simulink model "acf_rl_native"  (R2026b)
settings: Solver=ode4  StopTime=inf  FixedStep=3.3333333333333333e-06
InitFcn:
  | acf_select_actuator(bdroot);
model workspace (MAT data in the model file):
  acfControlVersion = 'force-observer-v1'
  acfImplementation = 'simple'
  acfLayoutVersion = 1
  p : object (value not decoded)
  pCompliant : object (value not decoded)
  pNearContact : object (value not decoded)
  pNoSprings : object (value not decoded)
  pRecommended : object (value not decoded)
symbols that are objects in the model workspace (value not decoded): p
undefined symbols (not defined in the file or in its folder): DiscIntNeverNeededParam
libraries: sl_discontinuities x1
(part 3 of 4)

== system acf_rl_native/Lateral B-S force measurement/Engineered common AA and EMA ==
  analog input : Inport
  ADC analog input filter : StateSpace  A=p.adcStudy.d.converterAnalog.A  B=p.adcStudy.d.converterAnalog.B  C=p.adcStudy.d.converterAnalog.C  D=p.adcStudy.d.converterAnalog.D  InitialCondition=((p.force.reference*(1+p.uncertainty.forceScaleX)*(-p.contact.mu*cos(p.uncertainty.forceFrameAngle_rad)-sin(p.uncertainty.forceFrameAngle_rad)+p.uncertainty.forceCrossXFromZ)))*p.adcStudy.d.converterAnalog.steadyStatePerUnitInput
  ADC clipping magnitude : Abs  SaturateOnIntegerOverflow=off
  ADC input and output noise : Sum
  ADC output noise correlation : DiscreteTransferFcn  Numerator=p.adcStudy.d.converterNoise.numerator  Denominator=p.adcStudy.d.converterNoise.denominator  SampleTime=p.adcStudy.outputSampleTime_s
  ADC range difference : Sum  Inputs=+-
  Actual ADC input range : Saturate  UpperLimit=p.adcStudy.forceAdcRange_N  LowerLimit=-(p.adcStudy.forceAdcRange_N)
  Actual ADC output samples : ZeroOrderHold  SampleTime=p.adcStudy.outputSampleTime_s
  Actual converter quantization : Quantizer  QuantizationInterval=max(p.adcStudy.forceQuantum_N,1e-15)
  Continuous analog front end : StateSpace  A=p.adcStudy.d.channels.lateral.analogA  B=p.adcStudy.d.channels.lateral.analogB  C=p.adcStudy.d.channels.lateral.analogC  D=p.adcStudy.d.channels.lateral.analogD  InitialCondition=((p.force.reference*(1+p.uncertainty.forceScaleX)*(-p.contact.mu*cos(p.uncertainty.forceFrameAngle_rad)-sin(p.uncertainty.forceFrameAngle_rad)+p.uncertainty.forceCrossXFromZ)))*p.adcStudy.d.channels.lateral.analogSteadyStatePerUnitInput
  Converter output noise RMS : Gain  Gain=p.adcStudy.forceAdcNoiseRms_N
  Fresh per-conversion EMA : DiscreteTransferFcn  Numerator=p.adcStudy.d.channels.lateral.emaNumerator  Denominator=p.adcStudy.d.channels.lateral.emaDenominator  InitialStates=(round((((p.force.reference*(1+p.uncertainty.forceScaleX)*(-p.contact.mu*cos(p.uncertainty.forceFrameAngle_rad)-sin(p.uncertainty.forceFrameAngle_rad)+p.uncertainty.forceCrossXFromZ)))+(p.adcStudy.d.lateralGravityOffset_N))/(max(p.adcStudy.forceQuantum_N,1e-15)))*(max(p.adcStudy.forceQuantum_N,1e-15))-round((p.adcStudy.d.lateralGravityOffset_N)/(max(p.adcStudy.forceQuantum_N,1e-15)))*(max(p.adcStudy.forceQuantum_N,1e-15)))*p.adcStudy.d.channels.lateral.emaSteadyStatePerUnitInput  SampleTime=p.adcStudy.outputSampleTime_s
  Independent converter output noise : RandomNumber  Seed=p.sensor.seed+2808  SampleTime=p.adcStudy.outputSampleTime_s
  Known quantized static offset : Bias  Bias=-round((p.adcStudy.d.lateralGravityOffset_N)/(max(p.adcStudy.forceQuantum_N,1e-15)))*(max(p.adcStudy.forceQuantum_N,1e-15))  SaturateOnIntegerOverflow=off
  Native converter impulse response : DiscreteTransferFcn  Numerator=p.adcStudy.d.converter.numerator  Denominator=p.adcStudy.d.converter.denominator  InitialStates=((p.force.reference*(1+p.uncertainty.forceScaleX)*(-p.contact.mu*cos(p.uncertainty.forceFrameAngle_rad)-sin(p.uncertainty.forceFrameAngle_rad)+p.uncertainty.forceCrossXFromZ)))*p.adcStudy.d.converter.steadyStatePerUnitInput  SampleTime=p.adcStudy.fineClock_s
  Restore physical static offset : Bias  Bias=p.adcStudy.d.lateralGravityOffset_N  SaturateOnIntegerOverflow=off
  conditioned output : Outport
  tag scope: lateral_adc_clip=global, lateral_adc_prequant=global
  wires:
  Actual ADC output samples/1 -> ADC input and output noise/1
  Independent converter output noise/1 -> Converter output noise RMS/1
  Converter output noise RMS/1 -> ADC output noise correlation/1
  ADC output noise correlation/1 -> ADC input and output noise/2
  ADC input and output noise/1 -> Restore physical static offset/1
  Restore physical static offset/1 -> Actual ADC input range/1, [lateral_adc_prequant], ADC range difference/1
  Actual ADC input range/1 -> Actual converter quantization/1, ADC range difference/2
  Actual converter quantization/1 -> Known quantized static offset/1
  ADC range difference/1 -> ADC clipping magnitude/1
  ADC clipping magnitude/1 -> [lateral_adc_clip]
  analog input/1 -> Continuous analog front end/1
  Continuous analog front end/1 -> ADC analog input filter/1
  ADC analog input filter/1 -> Native converter impulse response/1
  Native converter impulse response/1 -> Actual ADC output samples/1
  Known quantized static offset/1 -> Fresh per-conversion EMA/1
  Fresh per-conversion EMA/1 -> conditioned output/1

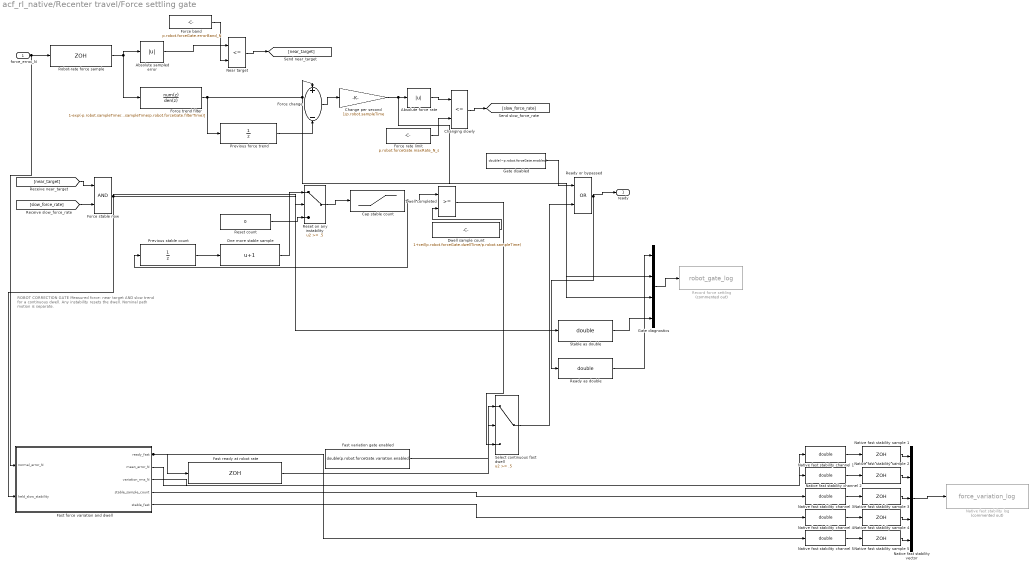
== system acf_rl_native/Recenter travel/Force settling gate ==
  note: ROBOT CORRECTION GATE
      | Measured force: near target AND slow trend for a continuous dwell.
      | Any instability resets the dwell. Nominal path motion is separate.
  force_error_N : Inport
  Absolute force rate : Abs  SaturateOnIntegerOverflow=off
  Absolute sampled error : Abs  SaturateOnIntegerOverflow=off
  Cap stable count : Saturate  UpperLimit=1+ceil(p.robot.forceGate.dwellTime/p.robot.sampleTime)  LowerLimit=0
  Change per second : Gain  Gain=1/p.robot.sampleTime
  Changing slowly : RelationalOperator  Operator=<=  OutDataTypeStr=boolean  RndMeth=Simplest  InputSameDT=off
  Dwell completed : RelationalOperator  OutDataTypeStr=boolean  RndMeth=Simplest  InputSameDT=off
  Dwell sample count : Constant  Value=1+ceil(p.robot.forceGate.dwellTime/p.robot.sampleTime)
  Fast force variation and dwell : Subsystem
  Fast ready at robot rate : ZeroOrderHold  SampleTime=p.robot.sampleTime
  Fast variation gate enabled : Constant  Value=double(p.robot.forceGate.variation.enabled)
  Force band : Constant  Value=p.robot.forceGate.errorBand_N
  Force change : Sum  Inputs=+-
  Force rate limit : Constant  Value=p.robot.forceGate.maxRate_N_s
  Force stable now : Logic  AllPortsSameDT=off  OutDataTypeStr=boolean
  Force trend filter : DiscreteTransferFcn  Numerator=1-exp(-p.robot.sampleTime/p.robot.forceGate.filterTime)  Denominator=[1 -exp(-p.robot.sampleTime/p.robot.forceGate.filterTime)]  SampleTime=p.robot.sampleTime
  Gate diagnostics : Mux
  Gate disabled : Constant  Value=double(~p.robot.forceGate.enabled)
  Native fast stability channel {1..5} (5 alike) : DataTypeConversion  OutDataTypeStr=double  SaturateOnIntegerOverflow=off  RndMeth=Floor
  Native fast stability log : ToWorkspace  Commented=on  VariableName=force_variation_log  SaveFormat=Timeseries  SampleTime=-1
  Native fast stability sample {1..5} (5 alike) : ZeroOrderHold  SampleTime=p.sim.step
  Native fast stability vector : Mux  Inputs=5
  Near target : RelationalOperator  Operator=<=  OutDataTypeStr=boolean  RndMeth=Simplest  InputSameDT=off
  One more stable sample : Bias  Bias=1  SaturateOnIntegerOverflow=off
  Previous force trend : UnitDelay  SampleTime=p.robot.sampleTime
  Previous stable count : UnitDelay  SampleTime=p.robot.sampleTime
  Ready as double : DataTypeConversion  OutDataTypeStr=double  SaturateOnIntegerOverflow=off  RndMeth=Floor
  Ready or bypassed : Logic  Operator=OR  AllPortsSameDT=off  OutDataTypeStr=boolean
  Record force settling : ToWorkspace  Commented=on  VariableName=robot_gate_log  SaveFormat=Timeseries  SampleTime=p.robot.sampleTime
  Reset count : Constant  Value=0
  Reset on any instability : Switch  Threshold=.5  SaturateOnIntegerOverflow=off  InputSameDT=off
  Robot-rate force sample : ZeroOrderHold  SampleTime=p.robot.sampleTime
  Select continuous fast dwell : Switch  Threshold=.5  SaturateOnIntegerOverflow=off  InputSameDT=off
  Stable as double : DataTypeConversion  OutDataTypeStr=double  SaturateOnIntegerOverflow=off  RndMeth=Floor
  ready : Outport
  wires:
  force_error_N/1 -> Robot-rate force sample/1, Fast force variation and dwell/1(normal_error_N)
  Robot-rate force sample/1 -> Absolute sampled error/1, Force trend filter/1
  Absolute sampled error/1 -> Near target/1
  Force band/1 -> Near target/2
  Near target/1 -> [near_target]
  Force trend filter/1 -> Force change/1, Gate diagnostics/2, Previous force trend/1
  Previous force trend/1 -> Force change/2
  Force change/1 -> Change per second/1
  Change per second/1 -> Absolute force rate/1, Gate diagnostics/3
  Absolute force rate/1 -> Changing slowly/1
  Force rate limit/1 -> Changing slowly/2
  Changing slowly/1 -> [slow_force_rate]
  [near_target] -> Force stable now/1
  [slow_force_rate] -> Force stable now/2
  Previous stable count/1 -> One more stable sample/1
  One more stable sample/1 -> Reset on any instability/1
  Force stable now/1 -> Reset on any instability/2, Stable as double/1, Fast force variation and dwell/2(held_slow_stability)
  Reset count/1 -> Reset on any instability/3
  Reset on any instability/1 -> Cap stable count/1
  Cap stable count/1 -> Previous stable count/1, Dwell completed/1
  Dwell sample count/1 -> Dwell completed/2
  Gate disabled/1 -> Ready or bypassed/1
  Ready or bypassed/1 -> ready/1, Ready as double/1
  Gate diagnostics/1 -> Record force settling/1
  Ready as double/1 -> Gate diagnostics/1
  Stable as double/1 -> Gate diagnostics/4
  Fast force variation and dwell/1(ready_fast) -> Fast ready at robot rate/1, Native fast stability channel 5/1
  Fast ready at robot rate/1 -> Select continuous fast dwell/1
  Fast variation gate enabled/1 -> Select continuous fast dwell/2
  Dwell completed/1 -> Select continuous fast dwell/3
  Select continuous fast dwell/1 -> Ready or bypassed/2
  Fast force variation and dwell/2(mean_error_N) -> Native fast stability channel 1/1
  Native fast stability channel 1/1 -> Native fast stability sample 1/1
  Native fast stability sample 1/1 -> Native fast stability vector/1
  Fast force variation and dwell/3(variation_rms_N) -> Native fast stability channel 2/1
  Native fast stability channel 2/1 -> Native fast stability sample 2/1
  Native fast stability sample 2/1 -> Native fast stability vector/2
  Fast force variation and dwell/4(stable_sample_count) -> Native fast stability channel 3/1
  Native fast stability channel 3/1 -> Native fast stability sample 3/1
  Native fast stability sample 3/1 -> Native fast stability vector/3
  Fast force variation and dwell/5(stable_fast) -> Native fast stability channel 4/1
  Native fast stability channel 4/1 -> Native fast stability sample 4/1
  Native fast stability sample 4/1 -> Native fast stability vector/4
  Native fast stability channel 5/1 -> Native fast stability sample 5/1
  Native fast stability sample 5/1 -> Native fast stability vector/5
  Native fast stability vector/1 -> Native fast stability log/1

== system acf_rl_native/S accelerometer and ADC/X engineered common AA and EMA ==
  analog input : Inport
  ADC analog input filter : StateSpace  A=p.adcStudy.d.converterAnalog.A  B=p.adcStudy.d.converterAnalog.B  C=p.adcStudy.d.converterAnalog.C  D=p.adcStudy.d.converterAnalog.D  InitialCondition=(((1+p.accel.scaleError)*(cos(p.uncertainty.accelFrameAngle_rad)*(p.mechanics.gravity*sin(p.mechanics.angle))-sin(p.uncertainty.accelFrameAngle_rad)*(p.d.g))))*p.adcStudy.d.converterAnalog.steadyStatePerUnitInput
  ADC clipping magnitude : Abs  SaturateOnIntegerOverflow=off
  ADC input and output noise : Sum
  ADC output noise correlation : DiscreteTransferFcn  Numerator=p.adcStudy.d.converterNoise.numerator  Denominator=p.adcStudy.d.converterNoise.denominator  SampleTime=p.adcStudy.outputSampleTime_s
  ADC range difference : Sum  Inputs=+-
  Actual ADC input range : Saturate  UpperLimit=min(p.adcStudy.accelerationAdcRange_g,p.accel.range_g)*p.mechanics.gravity  LowerLimit=-(min(p.adcStudy.accelerationAdcRange_g,p.accel.range_g)*p.mechanics.gravity)
  Actual ADC output samples : ZeroOrderHold  SampleTime=p.adcStudy.outputSampleTime_s
  Actual converter quantization : Quantizer  QuantizationInterval=max(p.adcStudy.accelerationQuantum_m_s2,1e-15)
  Continuous analog front end : StateSpace  A=p.adcStudy.d.channels.acceleration.analogA  B=p.adcStudy.d.channels.acceleration.analogB  C=p.adcStudy.d.channels.acceleration.analogC  D=p.adcStudy.d.channels.acceleration.analogD  InitialCondition=(((1+p.accel.scaleError)*(cos(p.uncertainty.accelFrameAngle_rad)*(p.mechanics.gravity*sin(p.mechanics.angle))-sin(p.uncertainty.accelFrameAngle_rad)*(p.d.g))))*p.adcStudy.d.channels.acceleration.analogSteadyStatePerUnitInput
  Converter output noise RMS : Gain  Gain=p.adcStudy.accelerationAdcNoiseRms_m_s2
  Fresh per-conversion EMA : DiscreteTransferFcn  Numerator=p.adcStudy.d.channels.acceleration.emaNumerator  Denominator=p.adcStudy.d.channels.acceleration.emaDenominator  InitialStates=(round(((((1+p.accel.scaleError)*(cos(p.uncertainty.accelFrameAngle_rad)*(p.mechanics.gravity*sin(p.mechanics.angle))-sin(p.uncertainty.accelFrameAngle_rad)*(p.d.g))))+(0))/(max(p.adcStudy.accelerationQuantum_m_s2,1e-15)))*(max(p.adcStudy.accelerationQuantum_m_s2,1e-15))-round((0)/(max(p.adcStudy.accelerationQuantum_m_s2,1e-15)))*(max(p.adcStudy.accelerationQuantum_m_s2,1e-15)))*p.adcStudy.d.channels.acceleration.emaSteadyStatePerUnitInput  SampleTime=p.adcStudy.outputSampleTime_s
  Independent converter output noise : RandomNumber  Seed=p.sensor.seed+3540  SampleTime=p.adcStudy.outputSampleTime_s
  Known quantized static offset : Bias  Bias=-round((0)/(max(p.adcStudy.accelerationQuantum_m_s2,1e-15)))*(max(p.adcStudy.accelerationQuantum_m_s2,1e-15))  SaturateOnIntegerOverflow=off
  Native converter impulse response : DiscreteTransferFcn  Numerator=p.adcStudy.d.converter.numerator  Denominator=p.adcStudy.d.converter.denominator  InitialStates=(((1+p.accel.scaleError)*(cos(p.uncertainty.accelFrameAngle_rad)*(p.mechanics.gravity*sin(p.mechanics.angle))-sin(p.uncertainty.accelFrameAngle_rad)*(p.d.g))))*p.adcStudy.d.converter.steadyStatePerUnitInput  SampleTime=p.adcStudy.fineClock_s
  Restore physical static offset : Bias  SaturateOnIntegerOverflow=off
  conditioned output : Outport
  tag scope: acceleration_x_adc_clip=global, acceleration_x_adc_prequant=global
  wires:
  Actual ADC output samples/1 -> ADC input and output noise/1
  Independent converter output noise/1 -> Converter output noise RMS/1
  Converter output noise RMS/1 -> ADC output noise correlation/1
  ADC output noise correlation/1 -> ADC input and output noise/2
  ADC input and output noise/1 -> Restore physical static offset/1
  Restore physical static offset/1 -> Actual ADC input range/1, [acceleration_x_adc_prequant], ADC range difference/1
  Actual ADC input range/1 -> Actual converter quantization/1, ADC range difference/2
  Actual converter quantization/1 -> Known quantized static offset/1
  ADC range difference/1 -> ADC clipping magnitude/1
  ADC clipping magnitude/1 -> [acceleration_x_adc_clip]
  analog input/1 -> Continuous analog front end/1
  Continuous analog front end/1 -> ADC analog input filter/1
  ADC analog input filter/1 -> Native converter impulse response/1
  Native converter impulse response/1 -> Actual ADC output samples/1
  Known quantized static offset/1 -> Fresh per-conversion EMA/1
  Fresh per-conversion EMA/1 -> conditioned output/1

== system acf_rl_native/S accelerometer and ADC/Z engineered common AA and EMA ==
  analog input : Inport
  ADC analog input filter : StateSpace  A=p.adcStudy.d.converterAnalog.A  B=p.adcStudy.d.converterAnalog.B  C=p.adcStudy.d.converterAnalog.C  D=p.adcStudy.d.converterAnalog.D  InitialCondition=(((1+p.accel.scaleError)*(cos(p.uncertainty.accelFrameAngle_rad)*(p.d.g)+sin(p.uncertainty.accelFrameAngle_rad)*(p.mechanics.gravity*sin(p.mechanics.angle)))))*p.adcStudy.d.converterAnalog.steadyStatePerUnitInput
  ADC clipping magnitude : Abs  SaturateOnIntegerOverflow=off
  ADC input and output noise : Sum
  ADC output noise correlation : DiscreteTransferFcn  Numerator=p.adcStudy.d.converterNoise.numerator  Denominator=p.adcStudy.d.converterNoise.denominator  SampleTime=p.adcStudy.outputSampleTime_s
  ADC range difference : Sum  Inputs=+-
  Actual ADC input range : Saturate  UpperLimit=min(p.adcStudy.accelerationAdcRange_g,p.accel.range_g)*p.mechanics.gravity  LowerLimit=-(min(p.adcStudy.accelerationAdcRange_g,p.accel.range_g)*p.mechanics.gravity)
  Actual ADC output samples : ZeroOrderHold  SampleTime=p.adcStudy.outputSampleTime_s
  Actual converter quantization : Quantizer  QuantizationInterval=max(p.adcStudy.accelerationQuantum_m_s2,1e-15)
  Continuous analog front end : StateSpace  A=p.adcStudy.d.channels.acceleration.analogA  B=p.adcStudy.d.channels.acceleration.analogB  C=p.adcStudy.d.channels.acceleration.analogC  D=p.adcStudy.d.channels.acceleration.analogD  InitialCondition=(((1+p.accel.scaleError)*(cos(p.uncertainty.accelFrameAngle_rad)*(p.d.g)+sin(p.uncertainty.accelFrameAngle_rad)*(p.mechanics.gravity*sin(p.mechanics.angle)))))*p.adcStudy.d.channels.acceleration.analogSteadyStatePerUnitInput
  Converter output noise RMS : Gain  Gain=p.adcStudy.accelerationAdcNoiseRms_m_s2
  Fresh per-conversion EMA : DiscreteTransferFcn  Numerator=p.adcStudy.d.channels.acceleration.emaNumerator  Denominator=p.adcStudy.d.channels.acceleration.emaDenominator  InitialStates=(round(((((1+p.accel.scaleError)*(cos(p.uncertainty.accelFrameAngle_rad)*(p.d.g)+sin(p.uncertainty.accelFrameAngle_rad)*(p.mechanics.gravity*sin(p.mechanics.angle)))))+(0))/(max(p.adcStudy.accelerationQuantum_m_s2,1e-15)))*(max(p.adcStudy.accelerationQuantum_m_s2,1e-15))-round((0)/(max(p.adcStudy.accelerationQuantum_m_s2,1e-15)))*(max(p.adcStudy.accelerationQuantum_m_s2,1e-15)))*p.adcStudy.d.channels.acceleration.emaSteadyStatePerUnitInput  SampleTime=p.adcStudy.outputSampleTime_s
  Independent converter output noise : RandomNumber  Seed=p.sensor.seed+3542  SampleTime=p.adcStudy.outputSampleTime_s
  Known quantized static offset : Bias  Bias=-round((0)/(max(p.adcStudy.accelerationQuantum_m_s2,1e-15)))*(max(p.adcStudy.accelerationQuantum_m_s2,1e-15))  SaturateOnIntegerOverflow=off
  Native converter impulse response : DiscreteTransferFcn  Numerator=p.adcStudy.d.converter.numerator  Denominator=p.adcStudy.d.converter.denominator  InitialStates=(((1+p.accel.scaleError)*(cos(p.uncertainty.accelFrameAngle_rad)*(p.d.g)+sin(p.uncertainty.accelFrameAngle_rad)*(p.mechanics.gravity*sin(p.mechanics.angle)))))*p.adcStudy.d.converter.steadyStatePerUnitInput  SampleTime=p.adcStudy.fineClock_s
  Restore physical static offset : Bias  SaturateOnIntegerOverflow=off
  conditioned output : Outport
  tag scope: acceleration_z_adc_clip=global, acceleration_z_adc_prequant=global
  wires:
  Actual ADC output samples/1 -> ADC input and output noise/1
  Independent converter output noise/1 -> Converter output noise RMS/1
  Converter output noise RMS/1 -> ADC output noise correlation/1
  ADC output noise correlation/1 -> ADC input and output noise/2
  ADC input and output noise/1 -> Restore physical static offset/1
  Restore physical static offset/1 -> Actual ADC input range/1, [acceleration_z_adc_prequant], ADC range difference/1
  Actual ADC input range/1 -> Actual converter quantization/1, ADC range difference/2
  Actual converter quantization/1 -> Known quantized static offset/1
  ADC range difference/1 -> ADC clipping magnitude/1
  ADC clipping magnitude/1 -> [acceleration_z_adc_clip]
  analog input/1 -> Continuous analog front end/1
  Continuous analog front end/1 -> ADC analog input filter/1
  ADC analog input filter/1 -> Native converter impulse response/1
  Native converter impulse response/1 -> Actual ADC output samples/1
  Known quantized static offset/1 -> Fresh per-conversion EMA/1
  Fresh per-conversion EMA/1 -> conditioned output/1

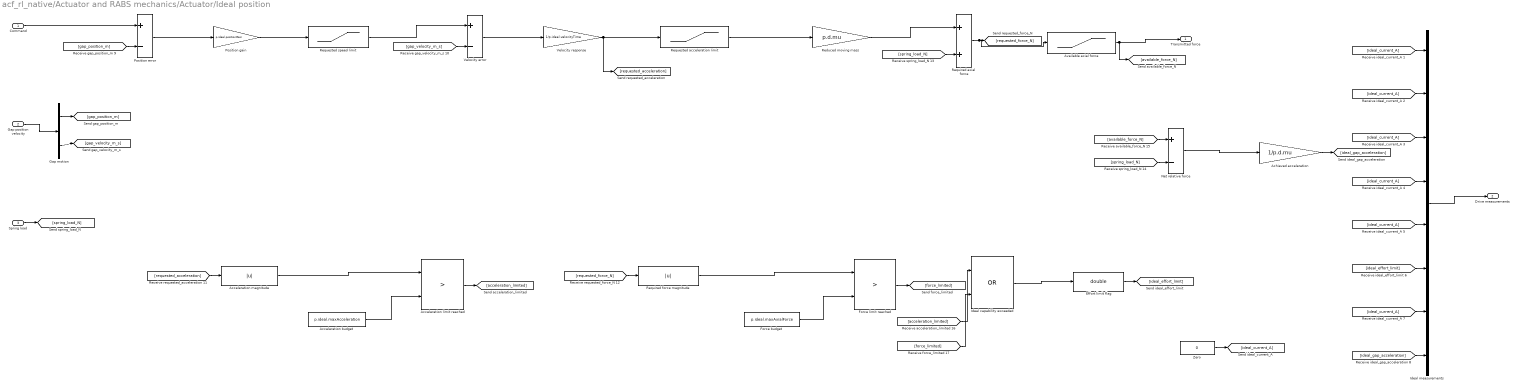
== system acf_rl_native/Actuator and RABS mechanics/Actuator/Ideal position ==
  Command : Inport
  Gap position velocity : Inport  Port=2
  Spring load : Inport  Port=3
  Acceleration budget : Constant  Value=p.ideal.maxAcceleration
  Acceleration limit reached : RelationalOperator  Operator=>  OutDataTypeStr=boolean  RndMeth=Simplest  InputSameDT=off
  Acceleration magnitude : Abs  SaturateOnIntegerOverflow=off
  Achieved acceleration : Gain  Gain=1/p.d.mu
  Available axial force : Saturate  UpperLimit=p.ideal.maxAxialForce  LowerLimit=-p.ideal.maxAxialForce
  Effort limit flag : DataTypeConversion  OutDataTypeStr=double  SaturateOnIntegerOverflow=off  RndMeth=Floor
  Force budget : Constant  Value=p.ideal.maxAxialForce
  Force limit reached : RelationalOperator  Operator=>  OutDataTypeStr=boolean  RndMeth=Simplest  InputSameDT=off
  Gap motion : Demux  Outputs=2
  Ideal capability exceeded : Logic  Operator=OR  AllPortsSameDT=off  OutDataTypeStr=boolean
  Ideal measurements : Mux  Inputs=8
  Net relative force : Sum  Inputs=+-
  Position error : Sum  Inputs=+-
  Position gain : Gain  Gain=p.ideal.positionGain
  Reduced moving mass : Gain  Gain=p.d.mu
  Requested acceleration limit : Saturate  UpperLimit=p.ideal.maxAcceleration  LowerLimit=-p.ideal.maxAcceleration
  Requested speed limit : Saturate  UpperLimit=p.ideal.maxSpeed  LowerLimit=-p.ideal.maxSpeed
  Required axial force : Sum
  Required force magnitude : Abs  SaturateOnIntegerOverflow=off
  Velocity error : Sum  Inputs=+-
  Velocity response : Gain  Gain=1/p.ideal.velocityTime
  Zero : Constant  Value=0
  Transmitted force : Outport
  Drive measurements : Outport  Port=2
  wires:
  Acceleration magnitude/1 -> Acceleration limit reached/1
  Acceleration budget/1 -> Acceleration limit reached/2
  [requested_acceleration] -> Acceleration magnitude/1
  Net relative force/1 -> Achieved acceleration/1
  Required axial force/1 -> Available axial force/1, [requested_force_N]
  Ideal capability exceeded/1 -> Effort limit flag/1
  Required force magnitude/1 -> Force limit reached/1
  Force budget/1 -> Force limit reached/2
  Gap position velocity/1 -> Gap motion/1
  [acceleration_limited] -> Ideal capability exceeded/1
  [force_limited] -> Ideal capability exceeded/2
  [ideal_current_A] -> Ideal measurements/1
  [ideal_current_A] -> Ideal measurements/2
  [ideal_current_A] -> Ideal measurements/3
  [ideal_current_A] -> Ideal measurements/4
  [ideal_current_A] -> Ideal measurements/5
  [ideal_effort_limit] -> Ideal measurements/6
  [ideal_current_A] -> Ideal measurements/7
  [ideal_gap_acceleration] -> Ideal measurements/8
  [available_force_N] -> Net relative force/1
  [spring_load_N] -> Net relative force/2
  Command/1 -> Position error/1
  [gap_position_m] -> Position error/2
  Position error/1 -> Position gain/1
  Requested acceleration limit/1 -> Reduced moving mass/1
  Velocity response/1 -> Requested acceleration limit/1, [requested_acceleration]
  Position gain/1 -> Requested speed limit/1
  Reduced moving mass/1 -> Required axial force/1
  [spring_load_N] -> Required axial force/2
  [requested_force_N] -> Required force magnitude/1
  Acceleration limit reached/1 -> [acceleration_limited]
  Available axial force/1 -> [available_force_N], Transmitted force/1
  Force limit reached/1 -> [force_limited]
  Gap motion/1 -> [gap_position_m]
  Gap motion/2 -> [gap_velocity_m_s]
  Zero/1 -> [ideal_current_A]
  Effort limit flag/1 -> [ideal_effort_limit]
  Achieved acceleration/1 -> [ideal_gap_acceleration]
  Spring load/1 -> [spring_load_N]
  Requested speed limit/1 -> Velocity error/1
  [gap_velocity_m_s] -> Velocity error/2
  Velocity error/1 -> Velocity response/1
  Ideal measurements/1 -> Drive measurements/1

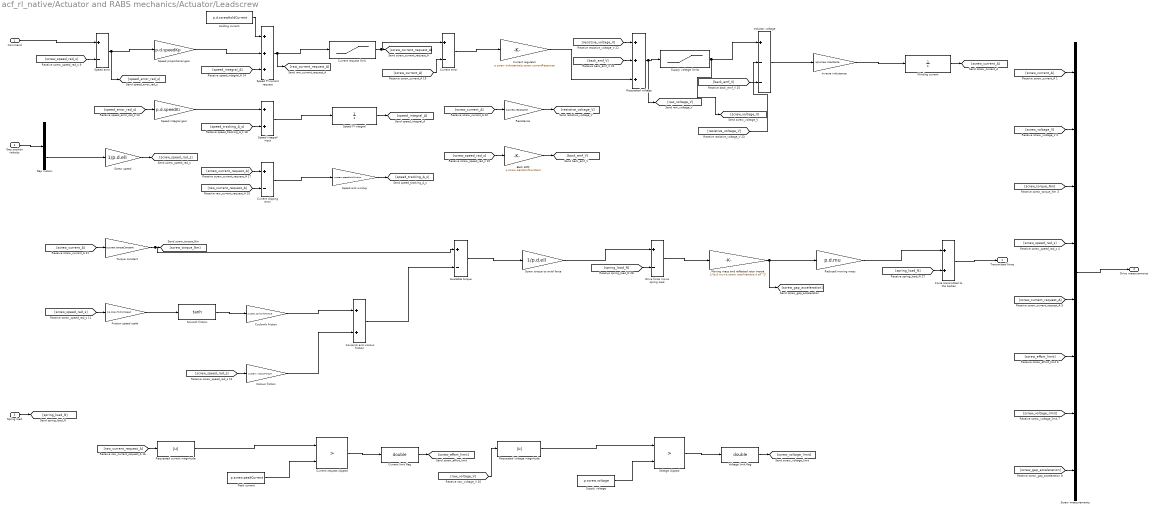
== system acf_rl_native/Actuator and RABS mechanics/Actuator/Leadscrew ==
  Command : Inport
  Gap position velocity : Inport  Port=2
  Spring load : Inport  Port=3
  Available torque : Sum  Inputs=+-
  Back EMF : Gain  Gain=p.screw.backEmfConstant
  Coulomb and viscous friction : Sum
  Coulomb friction : Gain  Gain=p.screw.coulombTorque
  Current clipping error : Sum  Inputs=+-
  Current error : Sum  Inputs=+-
  Current limit flag : DataTypeConversion  OutDataTypeStr=double  SaturateOnIntegerOverflow=off  RndMeth=Floor
  Current regulator : Gain  Gain=p.screw.inductance/p.screw.currentResponse
  Current request clipped : RelationalOperator  Operator=>  OutDataTypeStr=boolean  RndMeth=Simplest  InputSameDT=off
  Current request limit : Saturate  UpperLimit=p.screw.peakCurrent  LowerLimit=-p.screw.peakCurrent
  Drive force minus spring load : Sum  Inputs=+-
  Force transmitted to the bodies : Sum
  Friction speed scale : Gain  Gain=1/p.screw.frictionSpeed
  Gap motion : Demux  Outputs=2
  Holding current : Constant  Value=p.d.screwHoldCurrent
  Inductor voltage : Sum  Inputs=+--
  Inverse inductance : Gain  Gain=1/p.screw.inductance
  Moving mass and reflected rotor inertia : Gain  Gain=1/(p.d.mu+p.screw.rotorInertia/p.d.ell^2)
  Peak current : Constant  Value=p.screw.peakCurrent
  Reduced moving mass : Gain  Gain=p.d.mu
  Requested current magnitude : Abs  SaturateOnIntegerOverflow=off
  Requested voltage : Sum  Inputs=+++
  Requested voltage magnitude : Abs  SaturateOnIntegerOverflow=off
  Resistance : Gain  Gain=p.screw.resistance
  Screw measurements : Mux  Inputs=8
  Screw speed : Gain  Gain=1/p.d.ell
  Screw torque to axial force : Gain  Gain=1/p.d.ell
  Smooth friction : Trigonometry  Operator=tanh
  Speed PI current request : Sum  Inputs=+++
  Speed PI integral : Integrator
  Speed anti windup : Gain  Gain=p.screw.speedAntiWindup
  Speed error : Sum  Inputs=+-
  Speed integral gain : Gain  Gain=p.d.speedKi
  Speed integral input : Sum
  Speed proportional gain : Gain  Gain=p.d.speedKp
  Supply voltage : Constant  Value=p.screw.voltage
  Supply voltage limits : Saturate  UpperLimit=p.screw.voltage  LowerLimit=-p.screw.voltage
  Torque constant : Gain  Gain=p.screw.torqueConstant
  Viscous friction : Gain  Gain=p.screw.viscousTorque
  Voltage clipped : RelationalOperator  Operator=>  OutDataTypeStr=boolean  RndMeth=Simplest  InputSameDT=off
  Voltage limit flag : DataTypeConversion  OutDataTypeStr=double  SaturateOnIntegerOverflow=off  RndMeth=Floor
  Winding current : Integrator  InitialCondition=p.d.screwHoldCurrent
  Transmitted force : Outport
  Drive measurements : Outport  Port=2
  wires:
  Torque constant/1 -> Available torque/1, [screw_torque_Nm]
  Coulomb and viscous friction/1 -> Available torque/2
  [screw_speed_rad_s] -> Back EMF/1
  Coulomb friction/1 -> Coulomb and viscous friction/1
  Viscous friction/1 -> Coulomb and viscous friction/2
  Smooth friction/1 -> Coulomb friction/1
  [screw_current_request_A] -> Current clipping error/1
  [raw_current_request_A] -> Current clipping error/2
  Current request limit/1 -> Current error/1, [screw_current_request_A]
  [screw_current_A] -> Current error/2
  Current request clipped/1 -> Current limit flag/1
  Current error/1 -> Current regulator/1
  Requested current magnitude/1 -> Current request clipped/1
  Peak current/1 -> Current request clipped/2
  Speed PI current request/1 -> Current request limit/1, [raw_current_request_A]
  Screw torque to axial force/1 -> Drive force minus spring load/1
  [spring_load_N] -> Drive force minus spring load/2
  Reduced moving mass/1 -> Force transmitted to the bodies/1
  [spring_load_N] -> Force transmitted to the bodies/2
  [screw_speed_rad_s] -> Friction speed scale/1
  Gap position velocity/1 -> Gap motion/1
  Supply voltage limits/1 -> Inductor voltage/1, [screw_voltage_V]
  [resistive_voltage_V] -> Inductor voltage/2
  [back_emf_V] -> Inductor voltage/3
  Inductor voltage/1 -> Inverse inductance/1
  Drive force minus spring load/1 -> Moving mass and reflected rotor inertia/1
  Moving mass and reflected rotor inertia/1 -> Reduced moving mass/1, [screw_gap_acceleration]
  [raw_current_request_A] -> Requested current magnitude/1
  [resistive_voltage_V] -> Requested voltage/1
  [back_emf_V] -> Requested voltage/2
  Current regulator/1 -> Requested voltage/3
  [raw_voltage_V] -> Requested voltage magnitude/1
  [screw_current_A] -> Resistance/1
  [screw_current_A] -> Screw measurements/1
  [screw_voltage_V] -> Screw measurements/2
  [screw_torque_Nm] -> Screw measurements/3
  [screw_speed_rad_s] -> Screw measurements/4
  [screw_current_request_A] -> Screw measurements/5
  [screw_effort_limit] -> Screw measurements/6
  [screw_voltage_limit] -> Screw measurements/7
  [screw_gap_acceleration] -> Screw measurements/8
  Gap motion/2 -> Screw speed/1
  Available torque/1 -> Screw torque to axial force/1
  Back EMF/1 -> [back_emf_V]
  Requested voltage/1 -> [raw_voltage_V], Supply voltage limits/1
  Resistance/1 -> [resistive_voltage_V]
  Winding current/1 -> [screw_current_A]
  Current limit flag/1 -> [screw_effort_limit]
  Screw speed/1 -> [screw_speed_rad_s]
  Voltage limit flag/1 -> [screw_voltage_limit]
  Speed error/1 -> [speed_error_rad_s], Speed proportional gain/1
  Speed PI integral/1 -> [speed_integral_A]
  Speed anti windup/1 -> [speed_tracking_A_s]
  Spring load/1 -> [spring_load_N]
  Friction speed scale/1 -> Smooth friction/1
  Holding current/1 -> Speed PI current request/1
  Speed proportional gain/1 -> Speed PI current request/2
  [speed_integral_A] -> Speed PI current request/3
  Speed integral input/1 -> Speed PI integral/1
  Current clipping error/1 -> Speed anti windup/1
  Command/1 -> Speed error/1
  [screw_speed_rad_s] -> Speed error/2
  [speed_error_rad_s] -> Speed integral gain/1
  Speed integral gain/1 -> Speed integral input/1
  [speed_tracking_A_s] -> Speed integral input/2
  [screw_current_A] -> Torque constant/1
  [screw_speed_rad_s] -> Viscous friction/1
  Requested voltage magnitude/1 -> Voltage clipped/1
  Supply voltage/1 -> Voltage clipped/2
  Voltage clipped/1 -> Voltage limit flag/1
  Inverse inductance/1 -> Winding current/1
  Force transmitted to the bodies/1 -> Transmitted force/1
  Screw measurements/1 -> Drive measurements/1

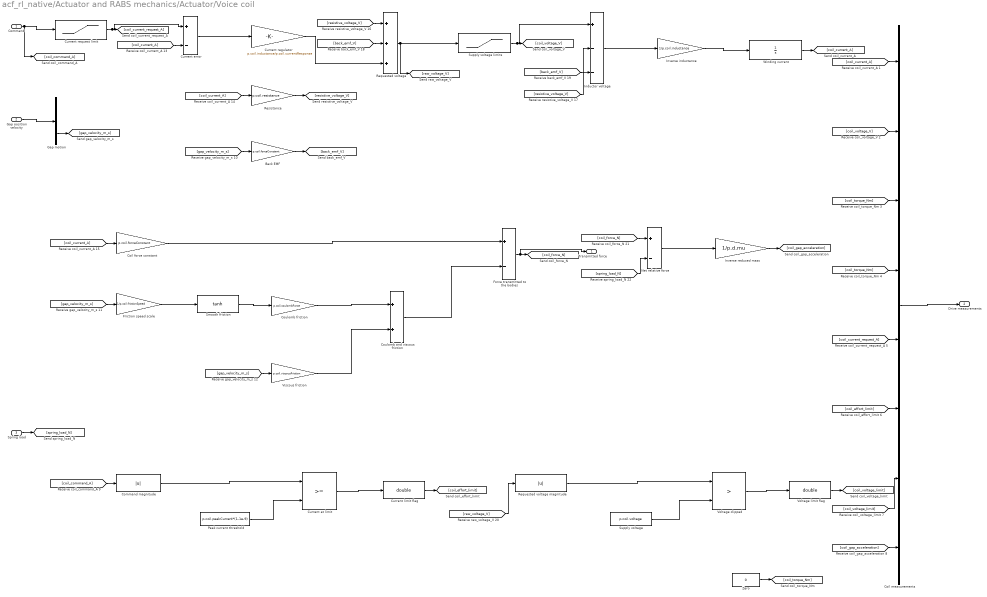
== system acf_rl_native/Actuator and RABS mechanics/Actuator/Voice coil ==
  Command : Inport
  Gap position velocity : Inport  Port=2
  Spring load : Inport  Port=3
  Back EMF : Gain  Gain=p.coil.forceConstant
  Coil force constant : Gain  Gain=p.coil.forceConstant
  Coil measurements : Mux  Inputs=8
  Command magnitude : Abs  SaturateOnIntegerOverflow=off
  Coulomb and viscous friction : Sum
  Coulomb friction : Gain  Gain=p.coil.coulombForce
  Current at limit : RelationalOperator  OutDataTypeStr=boolean  RndMeth=Simplest  InputSameDT=off
  Current error : Sum  Inputs=+-
  Current limit flag : DataTypeConversion  OutDataTypeStr=double  SaturateOnIntegerOverflow=off  RndMeth=Floor
  Current regulator : Gain  Gain=p.coil.inductance/p.coil.currentResponse
  Current request limit : Saturate  UpperLimit=p.coil.peakCurrent  LowerLimit=-p.coil.peakCurrent
  Force transmitted to the bodies : Sum  Inputs=+-
  Friction speed scale : Gain  Gain=1/p.coil.frictionSpeed
  Gap motion : Demux  Outputs=2
  Inductor voltage : Sum  Inputs=+--
  Inverse inductance : Gain  Gain=1/p.coil.inductance
  Inverse reduced mass : Gain  Gain=1/p.d.mu
  Net relative force : Sum  Inputs=+-
  Peak current threshold : Constant  Value=p.coil.peakCurrent*(1-1e-9)
  Requested voltage : Sum  Inputs=+++
  Requested voltage magnitude : Abs  SaturateOnIntegerOverflow=off
  Resistance : Gain  Gain=p.coil.resistance
  Smooth friction : Trigonometry  Operator=tanh
  Supply voltage : Constant  Value=p.coil.voltage
  Supply voltage limits : Saturate  UpperLimit=p.coil.voltage  LowerLimit=-p.coil.voltage
  Viscous friction : Gain  Gain=p.coil.viscousFriction
  Voltage clipped : RelationalOperator  Operator=>  OutDataTypeStr=boolean  RndMeth=Simplest  InputSameDT=off
  Voltage limit flag : DataTypeConversion  OutDataTypeStr=double  SaturateOnIntegerOverflow=off  RndMeth=Floor
  Winding current : Integrator  InitialCondition=p.d.coilHoldCurrent
  Zero : Constant  Value=0
  Transmitted force : Outport
  Drive measurements : Outport  Port=2
  wires:
  [gap_velocity_m_s] -> Back EMF/1
  [coil_current_A] -> Coil force constant/1
  [coil_current_A] -> Coil measurements/1
  [coil_voltage_V] -> Coil measurements/2
  [coil_torque_Nm] -> Coil measurements/3
  [coil_torque_Nm] -> Coil measurements/4
  [coil_current_request_A] -> Coil measurements/5
  [coil_effort_limit] -> Coil measurements/6
  [coil_voltage_limit] -> Coil measurements/7
  [coil_gap_acceleration] -> Coil measurements/8
  [coil_command_A] -> Command magnitude/1
  Coulomb friction/1 -> Coulomb and viscous friction/1
  Viscous friction/1 -> Coulomb and viscous friction/2
  Smooth friction/1 -> Coulomb friction/1
  Command magnitude/1 -> Current at limit/1
  Peak current threshold/1 -> Current at limit/2
  Current request limit/1 -> Current error/1, [coil_current_request_A]
  [coil_current_A] -> Current error/2
  Current at limit/1 -> Current limit flag/1
  Current error/1 -> Current regulator/1
  Command/1 -> Current request limit/1, [coil_command_A]
  Coil force constant/1 -> Force transmitted to the bodies/1
  Coulomb and viscous friction/1 -> Force transmitted to the bodies/2
  [gap_velocity_m_s] -> Friction speed scale/1
  Gap position velocity/1 -> Gap motion/1
  Supply voltage limits/1 -> Inductor voltage/1, [coil_voltage_V]
  [resistive_voltage_V] -> Inductor voltage/2
  [back_emf_V] -> Inductor voltage/3
  Inductor voltage/1 -> Inverse inductance/1
  Net relative force/1 -> Inverse reduced mass/1
  [coil_force_N] -> Net relative force/1
  [spring_load_N] -> Net relative force/2
  [resistive_voltage_V] -> Requested voltage/1
  [back_emf_V] -> Requested voltage/2
  Current regulator/1 -> Requested voltage/3
  [raw_voltage_V] -> Requested voltage magnitude/1
  [coil_current_A] -> Resistance/1
  Back EMF/1 -> [back_emf_V]
  Winding current/1 -> [coil_current_A]
  Current limit flag/1 -> [coil_effort_limit]
  Force transmitted to the bodies/1 -> [coil_force_N], Transmitted force/1
  Inverse reduced mass/1 -> [coil_gap_acceleration]
  Zero/1 -> [coil_torque_Nm]
  Voltage limit flag/1 -> [coil_voltage_limit]
  Gap motion/2 -> [gap_velocity_m_s]
  Requested voltage/1 -> [raw_voltage_V], Supply voltage limits/1
  Resistance/1 -> [resistive_voltage_V]
  Spring load/1 -> [spring_load_N]
  Friction speed scale/1 -> Smooth friction/1
  [gap_velocity_m_s] -> Viscous friction/1
  Requested voltage magnitude/1 -> Voltage clipped/1
  Supply voltage/1 -> Voltage clipped/2
  Voltage clipped/1 -> Voltage limit flag/1
  Inverse inductance/1 -> Winding current/1
  Coil measurements/1 -> Drive measurements/1

== system acf_rl_native/Contact force measurement/Head motion estimator/Issued force common ADC frame ==
  analog input : Inport
  ADC analog input filter : StateSpace  A=p.adcStudy.d.converterAnalog.A  B=p.adcStudy.d.converterAnalog.B  C=p.adcStudy.d.converterAnalog.C  D=p.adcStudy.d.converterAnalog.D  InitialCondition=(0)*p.adcStudy.d.converterAnalog.steadyStatePerUnitInput
  Actual ADC output samples : ZeroOrderHold  SampleTime=p.adcStudy.outputSampleTime_s
  Continuous analog front end : StateSpace  A=p.adcStudy.d.channels.frame.analogA  B=p.adcStudy.d.channels.frame.analogB  C=p.adcStudy.d.channels.frame.analogC  D=p.adcStudy.d.channels.frame.analogD  InitialCondition=(0)*p.adcStudy.d.channels.frame.analogSteadyStatePerUnitInput
  Fresh per-conversion EMA : DiscreteTransferFcn  Numerator=p.adcStudy.d.channels.frame.emaNumerator  Denominator=p.adcStudy.d.channels.frame.emaDenominator  InitialStates=(0)*p.adcStudy.d.channels.frame.emaSteadyStatePerUnitInput  SampleTime=p.adcStudy.outputSampleTime_s
  Native converter impulse response : DiscreteTransferFcn  Numerator=p.adcStudy.d.converter.numerator  Denominator=p.adcStudy.d.converter.denominator  InitialStates=(0)*p.adcStudy.d.converter.steadyStatePerUnitInput  SampleTime=p.adcStudy.fineClock_s
  conditioned output : Outport
  wires:
  Fresh per-conversion EMA/1 -> conditioned output/1
  Actual ADC output samples/1 -> Fresh per-conversion EMA/1
  Native converter impulse response/1 -> Actual ADC output samples/1
  ADC analog input filter/1 -> Native converter impulse response/1
  Continuous analog front end/1 -> ADC analog input filter/1
  analog input/1 -> Continuous analog front end/1

== system acf_rl_native/Contact force measurement/Head motion estimator/Position common AA and EMA ==
  analog input : Inport
  ADC analog input filter : StateSpace  A=p.adcStudy.d.converterAnalog.A  B=p.adcStudy.d.converterAnalog.B  C=p.adcStudy.d.converterAnalog.C  D=p.adcStudy.d.converterAnalog.D  InitialCondition=(0)*p.adcStudy.d.converterAnalog.steadyStatePerUnitInput
  Actual ADC output samples : ZeroOrderHold  SampleTime=p.adcStudy.outputSampleTime_s
  Continuous analog front end : StateSpace  A=p.adcStudy.d.channels.position.analogA  B=p.adcStudy.d.channels.position.analogB  C=p.adcStudy.d.channels.position.analogC  D=p.adcStudy.d.channels.position.analogD  InitialCondition=(0)*p.adcStudy.d.channels.position.analogSteadyStatePerUnitInput
  Fresh per-conversion EMA : DiscreteTransferFcn  Numerator=p.adcStudy.d.channels.position.emaNumerator  Denominator=p.adcStudy.d.channels.position.emaDenominator  InitialStates=(0)*p.adcStudy.d.channels.position.emaSteadyStatePerUnitInput  SampleTime=p.adcStudy.outputSampleTime_s
  Native converter impulse response : DiscreteTransferFcn  Numerator=p.adcStudy.d.converter.numerator  Denominator=p.adcStudy.d.converter.denominator  InitialStates=(0)*p.adcStudy.d.converter.steadyStatePerUnitInput  SampleTime=p.adcStudy.fineClock_s
  conditioned output : Outport
  wires:
  analog input/1 -> Continuous analog front end/1
  Continuous analog front end/1 -> ADC analog input filter/1
  ADC analog input filter/1 -> Native converter impulse response/1
  Native converter impulse response/1 -> Actual ADC output samples/1
  Actual ADC output samples/1 -> Fresh per-conversion EMA/1
  Fresh per-conversion EMA/1 -> conditioned output/1

== system acf_rl_native/Contact force measurement/Head motion estimator/Robot acceleration common AA and EMA ==
  analog input : Inport
  ADC analog input filter : StateSpace  A=p.adcStudy.d.converterAnalog.A  B=p.adcStudy.d.converterAnalog.B  C=p.adcStudy.d.converterAnalog.C  D=p.adcStudy.d.converterAnalog.D  InitialCondition=(0)*p.adcStudy.d.converterAnalog.steadyStatePerUnitInput
  Actual ADC output samples : ZeroOrderHold  SampleTime=p.adcStudy.outputSampleTime_s
  Continuous analog front end : StateSpace  A=p.adcStudy.d.channels.frame.analogA  B=p.adcStudy.d.channels.frame.analogB  C=p.adcStudy.d.channels.frame.analogC  D=p.adcStudy.d.channels.frame.analogD  InitialCondition=(0)*p.adcStudy.d.channels.frame.analogSteadyStatePerUnitInput
  Fresh per-conversion EMA : DiscreteTransferFcn  Numerator=p.adcStudy.d.channels.frame.emaNumerator  Denominator=p.adcStudy.d.channels.frame.emaDenominator  InitialStates=(0)*p.adcStudy.d.channels.frame.emaSteadyStatePerUnitInput  SampleTime=p.adcStudy.outputSampleTime_s
  Native converter impulse response : DiscreteTransferFcn  Numerator=p.adcStudy.d.converter.numerator  Denominator=p.adcStudy.d.converter.denominator  InitialStates=(0)*p.adcStudy.d.converter.steadyStatePerUnitInput  SampleTime=p.adcStudy.fineClock_s
  conditioned output : Outport
  wires:
  analog input/1 -> Continuous analog front end/1
  Continuous analog front end/1 -> ADC analog input filter/1
  ADC analog input filter/1 -> Native converter impulse response/1
  Native converter impulse response/1 -> Actual ADC output samples/1
  Actual ADC output samples/1 -> Fresh per-conversion EMA/1
  Fresh per-conversion EMA/1 -> conditioned output/1

== system acf_rl_native/Contact force measurement/Head motion estimator/Robot velocity common AA and EMA ==
  analog input : Inport
  ADC analog input filter : StateSpace  A=p.adcStudy.d.converterAnalog.A  B=p.adcStudy.d.converterAnalog.B  C=p.adcStudy.d.converterAnalog.C  D=p.adcStudy.d.converterAnalog.D  InitialCondition=(0)*p.adcStudy.d.converterAnalog.steadyStatePerUnitInput
  Actual ADC output samples : ZeroOrderHold  SampleTime=p.adcStudy.outputSampleTime_s
  Continuous analog front end : StateSpace  A=p.adcStudy.d.channels.frame.analogA  B=p.adcStudy.d.channels.frame.analogB  C=p.adcStudy.d.channels.frame.analogC  D=p.adcStudy.d.channels.frame.analogD  InitialCondition=(0)*p.adcStudy.d.channels.frame.analogSteadyStatePerUnitInput
  Fresh per-conversion EMA : DiscreteTransferFcn  Numerator=p.adcStudy.d.channels.frame.emaNumerator  Denominator=p.adcStudy.d.channels.frame.emaDenominator  InitialStates=(0)*p.adcStudy.d.channels.frame.emaSteadyStatePerUnitInput  SampleTime=p.adcStudy.outputSampleTime_s
  Native converter impulse response : DiscreteTransferFcn  Numerator=p.adcStudy.d.converter.numerator  Denominator=p.adcStudy.d.converter.denominator  InitialStates=(0)*p.adcStudy.d.converter.steadyStatePerUnitInput  SampleTime=p.adcStudy.fineClock_s
  conditioned output : Outport
  wires:
  analog input/1 -> Continuous analog front end/1
  Continuous analog front end/1 -> ADC analog input filter/1
  ADC analog input filter/1 -> Native converter impulse response/1
  Native converter impulse response/1 -> Actual ADC output samples/1
  Actual ADC output samples/1 -> Fresh per-conversion EMA/1
  Fresh per-conversion EMA/1 -> conditioned output/1

== system acf_rl_native/Contact force measurement/Normal force projection/Measured drag geometry ==
  reconstructed_Rz_N : Inport
  reconstructed_Rx_N : Inport  Port=2
  estimated_slope : Inport  Port=3
  estimated_normal_N : Inport  Port=4
  normalizer : Inport  Port=5
  Axial normal-force geometry factor : Bias  Bias=1  SaturateOnIntegerOverflow=off
  Bound signed drag ratio : Saturate  UpperLimit=1  LowerLimit=-1
  Drag correction sign : Gain  Gain=-1
  Drag estimate valid as double : DataTypeConversion  OutDataTypeStr=double  SaturateOnIntegerOverflow=off  RndMeth=Floor
  Estimated drag slope product : Product  Inputs=**
  Filtered measured drag ratio : Sum
  Force sufficient for drag estimate : RelationalOperator  Operator=>  OutDataTypeStr=boolean  RndMeth=Simplest  InputSameDT=off
  Guard projection denominator : Saturate  UpperLimit=inf  LowerLimit=p.contact.dragRatioMinForce_N
  Hold drag estimate below force guard : Switch  Threshold=.5  SaturateOnIntegerOverflow=off  InputSameDT=off
  Measured drag ratio : Product  Inputs=*/
  Minimum observable normal force : Constant  Value=p.contact.dragRatioMinForce_N
  New drag estimate weight : Gain  Gain=p.d.dragRatio.inputWeight
  Normal force reference : Gain  Gain=p.force.reference
  Normal projection denominator : Product  Inputs=**
  Previous drag estimate weight : Gain  Gain=p.d.dragRatio.memoryWeight
  Previous filtered drag ratio : UnitDelay  SampleTime=p.force.sampleTime
  Requested axial force from measured drag : Product  Inputs=*/
  Slope times axial reaction : Product  Inputs=**
  Tangential force numerator : Sum  Inputs=--
  requested_Rz_N : Outport
  filtered_drag_ratio : Outport  Port=2
  bounded_raw_drag_ratio : Outport  Port=3
  drag_estimate_valid : Outport  Port=4
  wires:
  reconstructed_Rz_N/1 -> Slope times axial reaction/1
  estimated_slope/1 -> Slope times axial reaction/2, Estimated drag slope product/2
  Slope times axial reaction/1 -> Tangential force numerator/1
  reconstructed_Rx_N/1 -> Tangential force numerator/2
  estimated_normal_N/1 -> Normal projection denominator/1, Force sufficient for drag estimate/1
  normalizer/1 -> Normal projection denominator/2, Requested axial force from measured drag/2
  Normal projection denominator/1 -> Guard projection denominator/1
  Guard projection denominator/1 -> Measured drag ratio/2
  Tangential force numerator/1 -> Measured drag ratio/1
  Measured drag ratio/1 -> Bound signed drag ratio/1
  Minimum observable normal force/1 -> Force sufficient for drag estimate/2
  Bound signed drag ratio/1 -> Hold drag estimate below force guard/1, bounded_raw_drag_ratio/1
  Force sufficient for drag estimate/1 -> Hold drag estimate below force guard/2, Drag estimate valid as double/1
  Previous filtered drag ratio/1 -> Hold drag estimate below force guard/3, Previous drag estimate weight/1
  Hold drag estimate below force guard/1 -> New drag estimate weight/1
  New drag estimate weight/1 -> Filtered measured drag ratio/1
  Previous drag estimate weight/1 -> Filtered measured drag ratio/2
  Filtered measured drag ratio/1 -> Previous filtered drag ratio/1, Estimated drag slope product/1, filtered_drag_ratio/1
  Estimated drag slope product/1 -> Drag correction sign/1
  Drag correction sign/1 -> Axial normal-force geometry factor/1
  Axial normal-force geometry factor/1 -> Normal force reference/1
  Normal force reference/1 -> Requested axial force from measured drag/1
  Requested axial force from measured drag/1 -> requested_Rz_N/1
  Drag estimate valid as double/1 -> drag_estimate_valid/1

== system acf_rl_native/Force controller/Coil PI and PID/Lower spring inverse feedforward ==
  Desired lower load deviation : Sum  Inputs=+-
  Full native inverse log : ToWorkspace  Commented=on  VariableName=lower_inverse_log  SaveFormat=Timeseries  SampleTime=-1
  Known downstream S inertia : Gain  Gain=p.sensor.distalMass_model_kg
  Native audit sampling : ZeroOrderHold  SampleTime=p.sim.step
  Native inverse audit : Mux
  Optional inverse feedforward scale : Gain  Gain=double(p.inertial.lowerLoadInverse.enabled)*p.inertial.lowerLoadInverse.scale
  Proper identified lower-link inverse : DiscreteTransferFcn  Numerator=p.inertial.lowerLoadInverse.numerator  Denominator=p.inertial.lowerLoadInverse.denominator  InitialStates=zeros(3,1)  SampleTime=p.force.sampleTime
  extra_current_A : Outport
  wires:
  [inertial_axial_reference_deviation_N] -> Desired lower load deviation/1, Native inverse audit/1
  [measured_S_acceleration_z] -> Known downstream S inertia/1
  Known downstream S inertia/1 -> Desired lower load deviation/2, Native inverse audit/2
  Desired lower load deviation/1 -> Proper identified lower-link inverse/1, Native inverse audit/3
  Proper identified lower-link inverse/1 -> Optional inverse feedforward scale/1
  Optional inverse feedforward scale/1 -> extra_current_A/1, Native inverse audit/4
  Native inverse audit/1 -> Native audit sampling/1
  Native audit sampling/1 -> Full native inverse log/1

== system acf_rl_native/Force controller/Coil PI and PID/Measured motion feedforward ==
  Acceleration FF audit native rate : ZeroOrderHold  SampleTime=p.sim.step
  Acceleration FF audit vector : Mux  Inputs=2
  Acceleration FF native log : ToWorkspace  Commented=on  VariableName=acceleration_feedforward_log  SaveFormat=Timeseries  SampleTime=-1
  Acceleration FF prediction time : Gain  Gain=p.inertial.accelerationPrediction_s
  Causal acceleration for current FF : Sum
  Filtered measured acceleration rate : DiscreteTransferFcn  Numerator=p.d.accelerationPrediction.derivativeNumerator  Denominator=p.d.accelerationPrediction.derivativeDenominator  SampleTime=p.force.sampleTime
  Geometry current feedforward : Gain  Gain=p.contact.geometryFeedforwardScale/p.coil.forceConstant
  Guide Coulomb friction current : Gain  Gain=p.inertial.guideFrictionFeedforwardScale*p.coil.coulombForce/p.coil.forceConstant
  Guide friction direction : Trigonometry  Operator=tanh
  Guide friction feedforward : Sum
  Guide friction velocity scale : Gain  Gain=1/p.coil.frictionSpeed
  Guide viscous friction current : Gain  Gain=p.inertial.guideFrictionFeedforwardScale*p.coil.viscousFriction/p.coil.forceConstant
  Identified guide prediction time : Gain  Gain=p.inertial.guideVelocityPrediction_s
  Measured acceleration current feedforward : Gain  Gain=-p.inertial.accelerationFeedforwardScale*(p.uncertainty.massB_model_kg+p.sensor.distalMass_model_kg)/p.uncertainty.forceConstant_model_N_A
  Measured head gap acceleration : Sum  Inputs=+-
  Predicted guide velocity : Sum
  acceleration_current_A : Outport
  geometry_current_A : Outport  Port=2
  friction_current_A : Outport  Port=3
  tag scope: upper_estimated_guide_friction_current=global
  wires:
  Guide friction feedforward/1 -> friction_current_A/1, [upper_estimated_guide_friction_current]
  Guide friction velocity scale/1 -> Guide friction direction/1
  [upper_estimated_A_acceleration_aligned] -> Measured head gap acceleration/1
  Measured acceleration current feedforward/1 -> acceleration_current_A/1
  Guide friction direction/1 -> Guide Coulomb friction current/1
  [inertial_axial_reference_deviation_N] -> Geometry current feedforward/1
  Guide Coulomb friction current/1 -> Guide friction feedforward/2
  Measured head gap acceleration/1 -> Identified guide prediction time/1
  Guide viscous friction current/1 -> Guide friction feedforward/1
  Geometry current feedforward/1 -> geometry_current_A/1
  [measured_S_acceleration_z] -> Measured head gap acceleration/2, Filtered measured acceleration rate/1, Causal acceleration for current FF/1, Acceleration FF audit vector/1
  Identified guide prediction time/1 -> Predicted guide velocity/2
  [inertial_head_gap_velocity] -> Predicted guide velocity/1
  Predicted guide velocity/1 -> Guide friction velocity scale/1, Guide viscous friction current/1
  Filtered measured acceleration rate/1 -> Acceleration FF prediction time/1
  Acceleration FF prediction time/1 -> Causal acceleration for current FF/2
  Causal acceleration for current FF/1 -> Measured acceleration current feedforward/1, Acceleration FF audit vector/2
  Acceleration FF audit vector/1 -> Acceleration FF audit native rate/1
  Acceleration FF audit native rate/1 -> Acceleration FF native log/1
